simulink model "aero2_motor_ip_R2021a"  (R2021a)
settings: Solver=ode1  StartTime=0.0  StopTime=1  FixedStep=0.002  RelTol=1e-3
model workspace (MAT data in the model file):
  Kaw = 20
  Ki = 1.84164606325
  Kp = 0.216370391856
  meas_on = 0
settings Model: Creator=matiasgarcia  LastModifiedBy=matiasgarcia
settings DataIOCC: SaveOutput=off  SignalLogging=off  SaveTime=off
settings DebuggingCC: UnconnectedInputMsg=none  UnconnectedOutputMsg=none  UnconnectedLineMsg=none
settings ModelReferenceCC: EnableRefExpFcnMdlSchedulingChecks=off
settings RTWCC: Description=Generic Real-Time Target  GPUComputeCapability=5.0  DLArmComputeVersion=20.02.1

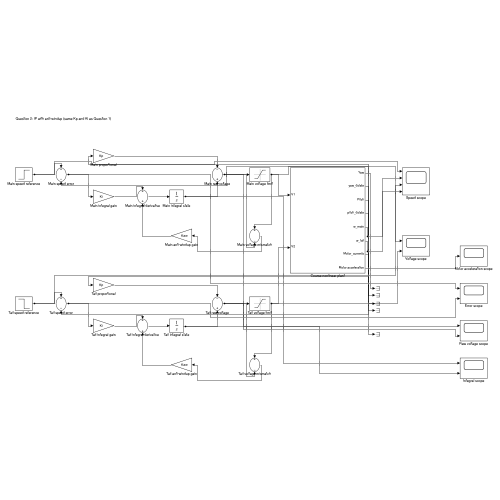
[thumbnail: Simulink's stored preview of the top-level diagram]
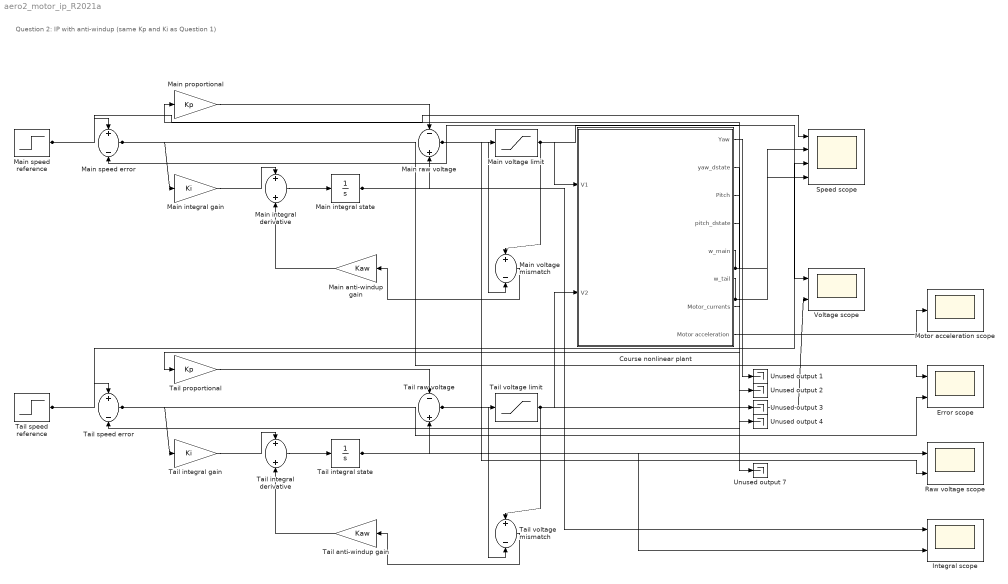
== system aero2_motor_ip_R2021a ==
  note: Question 2: IP with anti-windup (same Kp and Ki as Question 1)
  Course nonlinear plant : Subsystem  mask{meas=meas_on}
      mask prompts: meas "Measurement effects (1 = encoder quantization + sensor noise, 0 = ideal)"
      mask help: Simplified twin-rotor model (eq. (simp) of twin_rotor_FL_merged.tex) with DC-motor rotor dynamics. Inputs: V1 main-rotor voltage, V2 tail-rotor voltage [V]. Outputs: same signals as the QUARC interface of lin_feedback_v1.slx, continuous (no zero-order holds; sensor noise generated at Ts).
  Error scope : Scope  NumInputPorts=2
  Integral scope : Scope  NumInputPorts=2
  Main anti-windup gain : Gain  Gain=Kaw
  Main integral derivative : Sum
  Main integral gain : Gain  Gain=Ki
  Main integral state : Integrator
  Main proportional : Gain  Gain=Kp
  Main raw voltage : Sum  Inputs=-+
  Main speed error : Sum  Inputs=+-
  Main speed reference : Step  Time=0.1  After=100  SampleTime=0
  Main voltage limit : Saturate  UpperLimit=24  LowerLimit=-24
  Main voltage mismatch : Sum  Inputs=+-
  Motor acceleration scope : Scope
  Raw voltage scope : Scope  NumInputPorts=2
  Speed scope : Scope  NumInputPorts=4
  Tail anti-windup gain : Gain  Gain=Kaw
  Tail integral derivative : Sum
  Tail integral gain : Gain  Gain=Ki
  Tail integral state : Integrator
  Tail proportional : Gain  Gain=Kp
  Tail raw voltage : Sum  Inputs=-+
  Tail speed error : Sum  Inputs=+-
  Tail speed reference : Step  Time=0.1  After=-100  SampleTime=0
  Tail voltage limit : Saturate  UpperLimit=24  LowerLimit=-24
  Tail voltage mismatch : Sum  Inputs=+-
  Unused output {1..4,7} (5 alike) : Terminator
  Voltage scope : Scope  NumInputPorts=2
  wires:
  Main speed reference/1 -> Main speed error/1, Speed scope/1
  Course nonlinear plant/5(w_main) -> Main speed error/2, Main proportional/1, Speed scope/2
  Main speed error/1 -> Main integral gain/1, Error scope/1
  Main integral gain/1 -> Main integral derivative/1
  Main voltage limit/1 -> Main voltage mismatch/1, Course nonlinear plant/1(V1), Voltage scope/1
  Main raw voltage/1 -> Main voltage mismatch/2, Main voltage limit/1, Raw voltage scope/1
  Main voltage mismatch/1 -> Main anti-windup gain/1
  Main anti-windup gain/1 -> Main integral derivative/2
  Main integral derivative/1 -> Main integral state/1
  Main proportional/1 -> Main raw voltage/1
  Main integral state/1 -> Main raw voltage/2, Integral scope/1
  Tail speed reference/1 -> Tail speed error/1, Speed scope/3
  Course nonlinear plant/6(w_tail) -> Tail speed error/2, Tail proportional/1, Speed scope/4
  Tail speed error/1 -> Tail integral gain/1, Error scope/2
  Tail integral gain/1 -> Tail integral derivative/1
  Tail voltage limit/1 -> Tail voltage mismatch/1, Course nonlinear plant/2(V2), Voltage scope/2
  Tail raw voltage/1 -> Tail voltage mismatch/2, Tail voltage limit/1, Raw voltage scope/2
  Tail voltage mismatch/1 -> Tail anti-windup gain/1
  Tail anti-windup gain/1 -> Tail integral derivative/2
  Tail integral derivative/1 -> Tail integral state/1
  Tail proportional/1 -> Tail raw voltage/1
  Tail integral state/1 -> Tail raw voltage/2, Integral scope/2
  Course nonlinear plant/1(Yaw) -> Unused output 1/1
  Course nonlinear plant/2(yaw_dstate) -> Unused output 2/1
  Course nonlinear plant/3(Pitch) -> Unused output 3/1
  Course nonlinear plant/4(pitch_dstate) -> Unused output 4/1
  Course nonlinear plant/7(Motor_currents) -> Unused output 7/1
  Course nonlinear plant/8(Motor acceleration) -> Motor acceleration scope/1

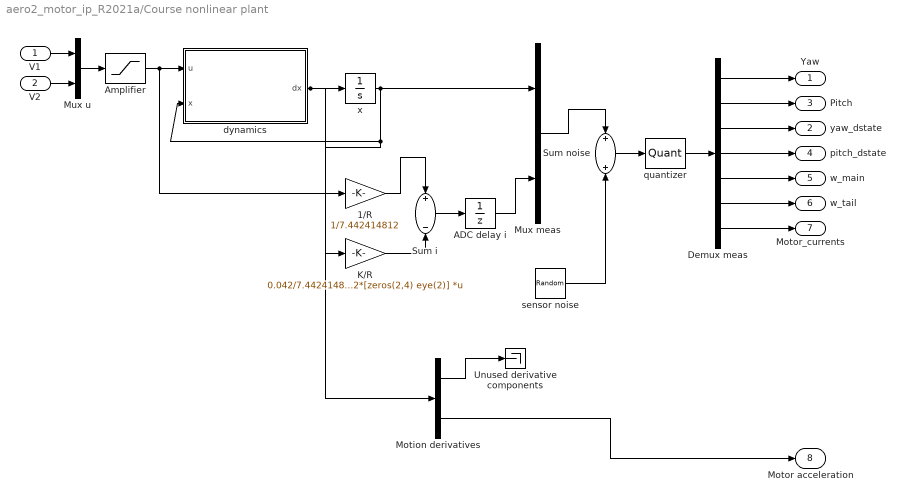
== system aero2_motor_ip_R2021a/Course nonlinear plant ==
  V1 : Inport
  V2 : Inport  Port=2
  1/R : Gain  Gain=1/7.442414812
  ADC delay i : UnitDelay  InitialCondition=[0;0]  SampleTime=0.002
  Amplifier : Saturate  UpperLimit=24  LowerLimit=-24
  Demux meas : Demux  Outputs=[1 1 1 1 1 1 2]
  K/R : Gain  Gain=0.042/7.442414812*[zeros(2,4) eye(2)]  Multiplication=Matrix(K*u)
  Motion derivatives : Demux  Outputs=[4 2]
  Mux meas : Mux  Inputs=[6 2]
  Mux u : Mux  Inputs=2
  Sum i : Sum  Inputs=+-
  Sum noise : Sum
  Unused derivative components : Terminator
  dynamics : MATLAB Function  TreatAsAtomicUnit=on
  quantizer : Quantizer  QuantizationInterval=max((meas)*[0.0015339807878856412;0.0030679615757712823;0.001;0.001;0.050000000000000003;0.050000000000000003;0.001;0.001], 1e-12)
  sensor noise : RandomNumber  Mean=zeros(8,1)  Variance=((meas)*[0.0005;0.0005;0.005;0.005;0.3;0.3;0.01;0.01]).^2  Seed=[61027;18839;4421;30893;23341;7781;51117;9013]  SampleTime=0.002
  x : Integrator  InitialCondition=zeros(6,1)
  Yaw : Outport
  yaw_dstate : Outport  Port=2
  Pitch : Outport  Port=3
  pitch_dstate : Outport  Port=4
  w_main : Outport  Port=5
  w_tail : Outport  Port=6
  Motor_currents : Outport  Port=7
  Motor acceleration : Outport  Port=8
  wires:
  Demux meas/7 -> Motor_currents/1
  Demux meas/6 -> w_tail/1
  Demux meas/5 -> w_main/1
  Demux meas/4 -> pitch_dstate/1
  Demux meas/2 -> Pitch/1
  Demux meas/3 -> yaw_dstate/1
  Demux meas/1 -> Yaw/1
  quantizer/1 -> Demux meas/1
  Sum noise/1 -> quantizer/1
  sensor noise/1 -> Sum noise/2
  Mux meas/1 -> Sum noise/1
  ADC delay i/1 -> Mux meas/2
  Sum i/1 -> ADC delay i/1
  K/R/1 -> Sum i/2
  1/R/1 -> Sum i/1
  x/1 -> K/R/1, dynamics/2(x), Mux meas/1
  dynamics/1(dx) -> x/1, Motion derivatives/1
  Amplifier/1 -> 1/R/1, dynamics/1(u)
  Mux u/1 -> Amplifier/1
  V2/1 -> Mux u/2
  V1/1 -> Mux u/1
  Motion derivatives/1 -> Unused derivative components/1
  Motion derivatives/2 -> Motor acceleration/1

== matlab function aero2_motor_ip_R2021a/Course nonlinear plant/dynamics ==
  data: u input; dx output; x input
function dx = fcn(u, x)
%% Simplified twin-rotor model of aero2_model.pdf (2-DOF body + first-order motors)
p = struct('Jph', 0.64070000000000005, ...
    'jph', 0.01, ...
    'Jth', 0.71640000000000004, ...
    'G', 0.025399999999999999, ...
    'kT', 4.2486999999999997e-06, ...
    'kF', 2.5525999999999999e-05, ...
    'L', 0.16700000000000001, ...
    'Cor', 0.63070000000000004, ...
    'Dph', 0, ...
    'Dth', 0, ...
    'aw', 5.7800000000000002, ...
    'bw', 96.531999999999996);
dx = tr_simp_dyn(x, u, p);
end

function dx = tr_simp_dyn(x, u, p)
%TR_SIMP_DYN  Simplified twin-rotor model with voltage inputs (aero2_model.pdf).
%   Body: reduced 2-DOF model, eq. (simp)
%     Mq(th) [ddpsi; ddth] + cq + Bq dq + gq = Gamma(th) [wm|wm|; wt|wt|]
%   with cq = [-Cor sin(2th) dth dpsi; 1/2 Cor sin(2th) dpsi^2]
%   (no gyroscopic coupling, no motor reaction channel, s_m=+1, s_t=-1).
%   Rotors: first-order motor model of the hand-out
%     dw = -aw w + bw v
%   State x = [psi, theta, dpsi, dtheta, wm, wt], input u = [Um, Ut].
%   p: Jph jph Jth Dph Dth Cor L G kF kT aw bw (psim of tr_instructor_params).

    th = x(2);  dps = x(3);  dth = x(4);
    c = cos(th);  s = sin(th);
    tau = [x(5)*abs(x(5)); x(6)*abs(x(6))];

    Ms  = [p.Jph*c^2 + p.jph*s^2, 0; 0, p.Jth];
    Cs  = [-p.Cor*sin(2*th)*dth*dps; 0.5*p.Cor*sin(2*th)*dps^2];
    Ds  = [p.Dph*dps; p.Dth*dth];
    Gs  = [0; p.G*s];
    Gam = [c 0; 0 1]*[-p.kT, p.L*p.kF; p.L*p.kF, p.kT];
    ddq = Ms\(Gam*tau - Cs - Ds - Gs);

    dw  = -p.aw*x(5:6) + p.bw*u(:);
    dx  = [x(3:4); ddq; dw];
end
